simulink library "ASEToolBox"  (R2025b)
settings: Solver=ode45  StartTime=0.0  StopTime=10.0  RelTol=1e-3  EnableMultiTasking=on
values from neighbouring files (symbols this model uses):
  dt = get_param(gcbh, 'g_output_datatype')    [maskSysComCallbacks_Receive.m]    (also in maskSysComCallbacks_Send.m = get_param(gcbh, 'g_input_datatype'))
undefined symbols (not defined in the file or in its folder): dCx, dCy, dCz, DiscIntNeverNeededParam, Discrete, dmassX, dmassY, dmassZ, dMx, dMy, dMz, dp, dp0, dp1, dp2, dp3, dspblkCoreblockFVToolHelper, gcbh, lmd_high, lmd_low, magnitude, Newton, p0, p1, p2, p3, p4, phi0, phi000, phi1, phi2, phi3, phi4, r1, r2, r3, r4, Raphson, theta0, theta1, theta2, theta3, theta4, Time, u0, u1, u2, u3, v0, v0_max, v0_min, v1, v111, v2, v222, v3, v333, v4, W1, w1 ... (+4)
libraries: simulink x38, etargetslib x28, simulink_extras x5, slpidlib x2, ctrlSharedLib x2, aerolibatmos2 x1, aerolibconvert2 x1, aerolibtransform2 x1, sharedtransform x1, dspstat3 x1, dspsolvers x1
(part 4 of 6)

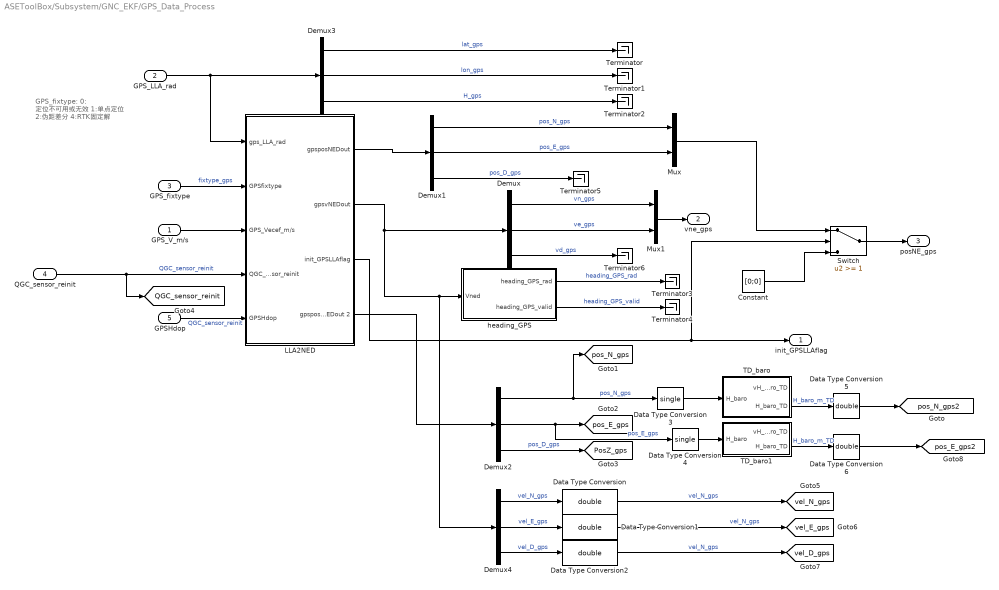
== system ASEToolBox/Subsystem/GNC_EKF/GPS_Data_Process ==
  note: GPS_fixtype:
      | 0: 定位不可用或无效
      | 1:单点定位
      | 2:伪距差分
      | 4:RTK固定解
  GPS_V_m/s : Inport
  GPS_LLA_rad : Inport  Port=2
  GPS_fixtype : Inport  Port=3
  QGC_sensor_reinit : Inport  Port=4
  GPSHdop : Inport  Port=5
  Constant : Constant  Value=[0;0]
  Data Type Conversion{,1..2,5..6} (5 alike) : DataTypeConversion  OutDataTypeStr=double  SaturateOnIntegerOverflow=off  RndMeth=Floor
  Data Type Conversion3 : DataTypeConversion  OutDataTypeStr=single  SaturateOnIntegerOverflow=off  RndMeth=Floor
  Data Type Conversion4 : DataTypeConversion  OutDataTypeStr=single  SaturateOnIntegerOverflow=off  RndMeth=Floor
  Demux{,1..4} (5 alike) : Demux  Outputs=3
  LLA2NED : Subsystem
  Mux : Mux  Inputs=2
  Mux1 : Mux  Inputs=2
  Switch : Switch  Threshold=1  SaturateOnIntegerOverflow=off  InputSameDT=off
  TD_baro : Subsystem
  TD_baro1 : Subsystem
  Terminator{,1..6} (7 alike) : Terminator
  heading_GPS : Subsystem
  init_GPSLLAflag : Outport
  vne_gps : Outport  Port=2
  posNE_gps : Outport  Port=3
  tag scope: PosZ_gps=global, QGC_sensor_reinit=global, pos_E_gps2=global, pos_E_gps=global, pos_N_gps2=global, pos_N_gps=global, vel_D_gps=global, vel_E_gps=global, vel_N_gps=global
  wires:
  GPS_fixtype/1 -> LLA2NED/2(GPSfixtype)  "fixtype_gps"
  Demux3/3 -> Terminator2/1  "H_gps"
  Demux/3 -> Terminator6/1  "vd_gps"
  Demux/1 -> Mux1/1  "vn_gps"
  GPS_LLA_rad/1 -> Demux3/1, LLA2NED/1(gps_LLA_rad)
  Demux/2 -> Mux1/2  "ve_gps"
  Demux3/2 -> Terminator1/1  "lon_gps"
  Demux3/1 -> Terminator/1  "lat_gps"
  QGC_sensor_reinit/1 -> [QGC_sensor_reinit], LLA2NED/4(QGC_sensor_reinit)  "QGC_sensor_reinit"
  LLA2NED/1("gpsposNEDout ") -> Demux1/1
  Demux1/1 -> Mux/1  "pos_N_gps"
  Demux1/2 -> Mux/2  "pos_E_gps"
  Demux1/3 -> Terminator5/1  "pos_D_gps"
  GPS_V_m/s/1 -> LLA2NED/3(GPS_Vecef_m/s)
  LLA2NED/2(gpsvNEDout) -> Demux4/1, heading_GPS/1(Vned), Demux/1
  heading_GPS/1(heading_GPS_rad) -> Terminator3/1  "heading_GPS_rad"
  heading_GPS/2(heading_GPS_valid) -> Terminator4/1  "heading_GPS_valid"
  Mux/1 -> Switch/1
  Mux1/1 -> vne_gps/1
  GPSHdop/1 -> LLA2NED/5(GPSHdop)  "QGC_sensor_reinit"
  LLA2NED/3(init_GPSLLAflag) -> Switch/2, init_GPSLLAflag/1
  Constant/1 -> Switch/3
  Switch/1 -> posNE_gps/1
  Demux2/1 -> [pos_N_gps], Data Type Conversion3/1  "pos_N_gps"
  Demux2/3 -> [PosZ_gps]  "pos_D_gps"
  Demux2/2 -> Data Type Conversion4/1, [pos_E_gps]  "pos_E_gps"
  LLA2NED/4(gpsposNEDout 2) -> Demux2/1
  Demux4/2 -> Data Type Conversion1/1  "vel_E_gps"
  Demux4/3 -> Data Type Conversion2/1  "vel_D_gps"
  Demux4/1 -> Data Type Conversion/1  "vel_N_gps"
  Data Type Conversion/1 -> [vel_N_gps]  "vel_N_gps"
  Data Type Conversion1/1 -> [vel_E_gps]  "vel_N_gps"
  Data Type Conversion2/1 -> [vel_D_gps]  "vel_N_gps"
  TD_baro/2(H_baro_TD) -> Data Type Conversion5/1  "H_baro_m_TD"
  TD_baro1/2(H_baro_TD) -> Data Type Conversion6/1  "H_baro_m_TD"
  Data Type Conversion3/1 -> TD_baro/1(H_baro)
  Data Type Conversion4/1 -> TD_baro1/1(H_baro)
  Data Type Conversion5/1 -> [pos_N_gps2]
  Data Type Conversion6/1 -> [pos_E_gps2]

== system ASEToolBox/Subsystem/GNC_EKF/Translation_estimate ==
  Cbn : Inport
  accl_ned_m/s2 : Inport  Port=2
  vne_gps : Inport  Port=3
  posNE_gps1 : Inport  Port=4
  GPSstate : Inport  Port=5
  GPSHdop : Inport  Port=6
  QGC_init : Inport  Port=7
  Enable : EnablePort
  Subsystem : Subsystem
  Subsystem2 : Subsystem
  V_Horizontal_estimation1 : Subsystem  Commented=on
  translate to N : Subsystem
  vxy_estimout : Outport
  Pxy_estimout : Outport  Port=2
  wires:
  Cbn/1 -> translate to N/1(Cbn)
  accl_ned_m/s2/1 -> translate to N/2(accl_ned)
  QGC_init/1 -> Subsystem/4(QGC_init), Subsystem2/3(QGC_init)
  posNE_gps1/1 -> Subsystem/2(pxy_GPS)
  GPSHdop/1 -> Subsystem2/4(DOP), Subsystem/5(DOP)
  Subsystem/1(pxy_est) -> Pxy_estimout/1
  Subsystem2/1(vxy_est) -> vxy_estimout/1, Subsystem/1(vxy)
  translate to N/1(accel_Horizontal_predict) -> Subsystem2/1(axy)
  vne_gps/1 -> Subsystem2/2(vxy_GPS)
  Subsystem2/2(GPSv_enable) -> Subsystem/3(GPSv_enable)

== system ASEToolBox/ACEModule/IMU/Subsystem5/Subsystem ==
  In1 : Inport
  Enable : EnablePort
  Byte Unpack1 : etargetslib/Byte Unpack  dimensions={6}  datatypes={'single'}  byteAlign=1
      settings: LibrarySourceBlock=embeddedtargetslib/Host Communication/Byte Unpack
  Out1 : Outport
  wires:
  In1/1 -> Byte Unpack1/1
  Byte Unpack1/1 -> Out1/1

== system ASEToolBox/ACEModule/ServoCardUnpack/Subsystem6/Subsystem ==
  In1 : Inport
  Enable : EnablePort
  Byte Unpack1 : etargetslib/Byte Unpack  dimensions={7}  datatypes={'single'}  byteAlign=1
      settings: LibrarySourceBlock=embeddedtargetslib/Host Communication/Byte Unpack
  Out1 : Outport
  wires:
  In1/1 -> Byte Unpack1/1
  Byte Unpack1/1 -> Out1/1

== system ASEToolBox/Aerocraft Model/ACE Equation of 6DOF's Motion/ACE Centroid Motion/231 Motion Subsystem ==
  F_All/m : Inport
  Deal with zero1 : Subsystem
  Deal with zero2 : Subsystem
  Deal with zero3 : Subsystem
  Demux1 : Demux  Outputs=3
  Discrete-Time Integrator : DiscreteIntegrator  InitialCondition=17.45  SampleTime=-1  ICPrevOutput=DiscIntNeverNeededParam  ICPrevScaledInput=DiscIntNeverNeededParam
  Discrete-Time Integrator1 : DiscreteIntegrator  SampleTime=-1  ICPrevOutput=DiscIntNeverNeededParam  ICPrevScaledInput=DiscIntNeverNeededParam
  Discrete-Time Integrator2 : DiscreteIntegrator  InitialCondition=60*pi/180  SampleTime=-1  ICPrevOutput=DiscIntNeverNeededParam  ICPrevScaledInput=DiscIntNeverNeededParam
  Gain6 : Gain  Gain=-1
  Integrator1 : Integrator  Commented=on  InitialCondition=17.45
  Integrator2 : Integrator  Commented=on  InitialCondition=60*pi/180
  Integrator3 : Integrator  Commented=on
  Product8 : Product  Inputs=/*  SaturateOnIntegerOverflow=on  OutDataTypeStr=Inherit: Same as first input
  Product9 : Product  Inputs=//*  SaturateOnIntegerOverflow=on  OutDataTypeStr=Inherit: Same as first input
  cosine1 : Trigonometry  Operator=cos
  V : Outport
  theta : Outport  Port=2
  sigma : Outport  Port=3
  wires:
  Discrete-Time Integrator1/1 -> sigma/1
  Discrete-Time Integrator2/1 -> cosine1/1, theta/1
  Discrete-Time Integrator/1 -> V/1, Deal with zero3/1(In1), Deal with zero1/1(In1)
  Gain6/1 -> Product9/3
  Deal with zero3/1(Out1) -> Product9/2
  Deal with zero2/1(Out1) -> Product9/1
  Product8/1 -> Discrete-Time Integrator2/1
  F_All/m/1 -> Demux1/1
  Demux1/1 -> Discrete-Time Integrator/1
  Demux1/3 -> Gain6/1
  Product9/1 -> Discrete-Time Integrator1/1
  Demux1/2 -> Product8/2
  cosine1/1 -> Deal with zero2/1(In1)
  Deal with zero1/1(Out1) -> Product8/1

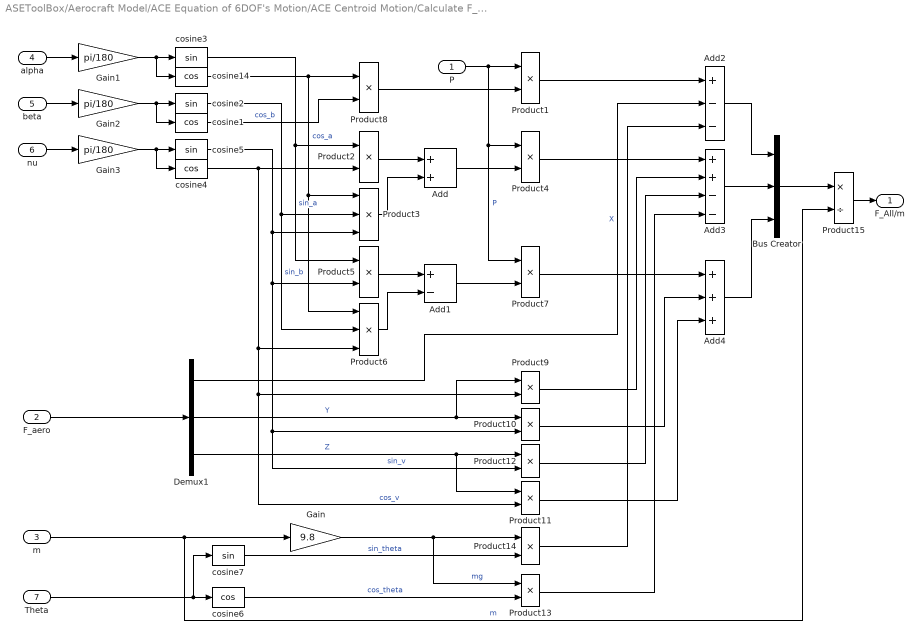
== system ASEToolBox/Aerocraft Model/ACE Equation of 6DOF's Motion/ACE Centroid Motion/Calculate F_all ==
  P : Inport
  F_aero : Inport  Port=2
  m : Inport  Port=3
  alpha : Inport  Port=4
  beta : Inport  Port=5
  nu : Inport  Port=6
  Theta : Inport  Port=7
  Add : Sum
  Add1 : Sum  Inputs=+-
  Add2 : Sum  Inputs=+--
  Add3 : Sum  Inputs=++--
  Add4 : Sum  Inputs=+++
  Bus Creator : BusCreator  Inputs=3
  Demux1 : Demux  Outputs=3
  Gain : Gain  Gain=9.8
  Gain1 : Gain  Gain=pi/180
  Gain2 : Gain  Gain=pi/180
  Gain3 : Gain  Gain=pi/180
  Product{1..2,4..5,7..14} (12 alike) : Product  Inputs=**  SaturateOnIntegerOverflow=on  OutDataTypeStr=Inherit: Same as first input
  Product15 : Product  Inputs=*/  SaturateOnIntegerOverflow=on  OutDataTypeStr=Inherit: Same as first input
  Product3 : Product  Inputs=***  SaturateOnIntegerOverflow=on  OutDataTypeStr=Inherit: Same as first input
  Product6 : Product  Inputs=***  SaturateOnIntegerOverflow=on  OutDataTypeStr=Inherit: Same as first input
  cosine{1,4,6,14} (4 alike) : Trigonometry  Operator=cos
  cosine{2..3,5,7} (4 alike) : Trigonometry
  F_All/m : Outport
  wires:
  F_aero/1 -> Demux1/1
  alpha/1 -> Gain1/1
  beta/1 -> Gain2/1
  nu/1 -> Gain3/1
  cosine14/1 -> Product8/1, Product3/1, Product6/1  "cos_a"
  cosine1/1 -> Product8/2  "cos_b"
  Product8/1 -> Product1/2
  P/1 -> Product1/1, Product4/1, Product7/1  "P"
  cosine4/1 -> Product2/2, Product6/3, Product9/2, Product11/2  "cos_v"
  cosine3/1 -> Product2/1, Product5/1  "sin_a"
  cosine2/1 -> Product3/2, Product6/2  "sin_b"
  cosine5/1 -> Product3/3, Product5/2, Product10/2, Product12/2  "sin_v"
  Product2/1 -> Add/1
  Product3/1 -> Add/2
  Add/1 -> Product4/2
  Product5/1 -> Add1/1
  Product6/1 -> Add1/2
  Add1/1 -> Product7/2
  Demux1/2 -> Product9/1, Product10/1  "Y"
  Demux1/3 -> Product12/1, Product11/1  "Z"
  m/1 -> Gain/1, Product15/2  "m"
  cosine7/1 -> Product14/2  "sin_theta"
  cosine6/1 -> Product13/2  "cos_theta"
  Product1/1 -> Add2/1
  Demux1/1 -> Add2/2  "X"
  Product14/1 -> Add2/3
  Product4/1 -> Add3/1
  Product9/1 -> Add3/2
  Product12/1 -> Add3/3
  Product13/1 -> Add3/4
  Product7/1 -> Add4/1
  Gain/1 -> Product14/1, Product13/1  "mg"
  Product10/1 -> Add4/2
  Product11/1 -> Add4/3
  Add2/1 -> Bus Creator/1
  Add3/1 -> Bus Creator/2
  Add4/1 -> Bus Creator/3
  Bus Creator/1 -> Product15/1
  Product15/1 -> F_All/m/1
  Theta/1 -> cosine6/1, cosine7/1
  Gain1/1 -> cosine3/1, cosine14/1
  Gain2/1 -> cosine2/1, cosine1/1
  Gain3/1 -> cosine5/1, cosine4/1

== system ASEToolBox/Aerocraft Model/ACE Equation of 6DOF's Motion/ACE Centroid Motion/Calculate xyz ==
  V : Inport
  theta : Inport  Port=2
  sigma : Inport  Port=3
  Discrete-Time Integrator : DiscreteIntegrator  SampleTime=-1  ICPrevOutput=DiscIntNeverNeededParam  ICPrevScaledInput=DiscIntNeverNeededParam
  Discrete-Time Integrator1 : DiscreteIntegrator  InitialCondition=0.001  SampleTime=-1  ICPrevOutput=DiscIntNeverNeededParam  ICPrevScaledInput=DiscIntNeverNeededParam
  Discrete-Time Integrator2 : DiscreteIntegrator  SampleTime=-1  ICPrevOutput=DiscIntNeverNeededParam  ICPrevScaledInput=DiscIntNeverNeededParam
  Mux1 : Mux  Inputs=3
  Mux2 : Mux  Inputs=3
  Vx : Product  Inputs=***  SaturateOnIntegerOverflow=on  OutDataTypeStr=Inherit: Same as first input
  Vy : Product  Inputs=**  SaturateOnIntegerOverflow=on  OutDataTypeStr=Inherit: Same as first input
  Vz : Gain  Gain=-1
  Vz. : Product  Inputs=***  SaturateOnIntegerOverflow=on  OutDataTypeStr=Inherit: Same as first input
  cosine10 : Trigonometry
  cosine11 : Trigonometry  Operator=cos
  cosine12 : Trigonometry  Operator=cos
  cosine14 : Trigonometry  Operator=cos
  cosine3 : Trigonometry
  x1 : Integrator  Commented=on
  y1 : Integrator  Commented=on  InitialCondition=0.001
  z1 : Integrator  Commented=on
  Vxyz : Outport
  xyz : Outport  Port=2
  wires:
  Discrete-Time Integrator2/1 -> Mux2/3
  Discrete-Time Integrator1/1 -> Mux2/2
  Discrete-Time Integrator/1 -> Mux2/1
  cosine10/1 -> Vz./3
  cosine14/1 -> Vz./2
  Vz/1 -> Mux1/3, Discrete-Time Integrator2/1  "vz"
  Vz./1 -> Vz/1
  Vy/1 -> Mux1/2, Discrete-Time Integrator1/1  "vy"
  Vx/1 -> Mux1/1, Discrete-Time Integrator/1  "vx"
  V/1 -> Vz./1, Vy/1, Vx/1
  Mux2/1 -> xyz/1
  Mux1/1 -> Vxyz/1
  cosine12/1 -> Vx/2
  cosine11/1 -> Vx/3
  cosine3/1 -> Vy/2
  theta/1 -> cosine14/1, cosine3/1, cosine11/1  "rad"
  sigma/1 -> cosine10/1, cosine12/1  "rad"

== system ASEToolBox/Aerocraft Model/ACE Equation of 6DOF's Motion/ACE Rotation Motion/Attitude Dynamic  ==
  note: d( w_x ) = M_x + (I_y-I_z)*w_y*w_z)
      |
      |  / I_x
      | .
  note: d( w_y ) = M_y + (I_z-I_x)*w_x*w_z)
      |
      |  / I_y
      | .
  note: d( w_z ) = M_z + (I_x-I_y)*w_x*w_y)
      |
      |  / I_z
      | .
  note: rad/s
  Mxyz : Inport
  Ixyz : Inport  Port=2
  Mux8 : Mux  Inputs=3
  Omega_Tx1 Subsystem : Subsystem
  Omega_Tx1 Subsystem1 : Subsystem
  Omega_Tx1 Subsystem2 : Subsystem
  Wxyz : Outport
  wires:
  Mxyz/1 -> Omega_Tx1 Subsystem/3(Mxyz), Omega_Tx1 Subsystem1/3(Mxyz), Omega_Tx1 Subsystem2/3(Mxyz)
  Mux8/1 -> Wxyz/1, Omega_Tx1 Subsystem/1(Wxyz), Omega_Tx1 Subsystem1/1(Wxyz), Omega_Tx1 Subsystem2/1(Wxyz)
  Omega_Tx1 Subsystem/1(Wx) -> Mux8/1
  Omega_Tx1 Subsystem1/1(Wy) -> Mux8/2
  Omega_Tx1 Subsystem2/1(Wz) -> Mux8/3
  Ixyz/1 -> Omega_Tx1 Subsystem/2(Ixyz), Omega_Tx1 Subsystem1/2(Ixyz), Omega_Tx1 Subsystem2/2(Ixyz)

== system ASEToolBox/Aerocraft Model/ACE Equation of 6DOF's Motion/ACE Rotation Motion/calculate Eular 231 ==
  note: d \phi = W_y * sin \gamma + W_z * cos \gamma
      |
      | d \psi = (W_y * cos \gamma - W_z * sin \gamma ) / cos \phi
      |
      | d \gamma = W_x  - tan \phi * ( W_y * cos \gamma - W_z * sin \gamma )
  Wxyz : Inport
  Eular0(deg) : Inport  Port=2
  Gain1 : Gain  Gain=pi/180
  Mux1 : Mux  Inputs=3
  PhiPsiGam : Gain  Gain=180/pi
  gam Subsystem : Subsystem
  phi Subsystem : Subsystem
  psi Subsystem : Subsystem
  Eular(deg) : Outport
  wires:
  Gain1/1 -> phi Subsystem/3(Eular0), psi Subsystem/3(Eular0), gam Subsystem/3(Eular0)
  PhiPsiGam/1 -> Eular(deg)/1
  Eular0(deg)/1 -> Gain1/1
  Mux1/1 -> PhiPsiGam/1, gam Subsystem/1(Eular), psi Subsystem/1(Eular), phi Subsystem/1(Eular)
  gam Subsystem/1(gam) -> Mux1/3
  psi Subsystem/1(psi) -> Mux1/2
  Wxyz/1 -> gam Subsystem/2(Wxyz), psi Subsystem/2(Wxyz), phi Subsystem/2(Wxyz)
  phi Subsystem/1(phi) -> Mux1/1

== system ASEToolBox/Aerocraft Model/ACE Equation of 6DOF's Motion/Aero Force & Moment/ACE Aerodynamic for 6DOF ==
  Ma : Inport
  abv : Inport  Port=2
  WXYZ : Inport  Port=3
  DeltXYZ : Inport  Port=4
  CD : Lookup2D  RowIndex=[-2 -1 0.5 1 2 3 4 5 6 7 8 9 10]  ColumnIndex=[0.3 0.4 0.5 0.6 0.7 0.8]  Table=|  SaturateOnIntegerOverflow=off  InputSameDT=off
      | [0.184400000000000	0.176300000000000	0.168500000000000	0.162600000000000	0.158700000000000	0.154800000000000
      | 0.194000000000000	0.185600000000000	0.177400000000000	0.171100000000000	0.166800000000000	0.162200000000000
      | 0.196300000000000	0.187800000000000	0.179600000000000	0.173200000000000	0.168700000000000	0.164000000000000
      | 0.194000000000000	0.185600000000000	0.177400000000000	0.171100000000000	0.166800000000000	0.162200000000000
      | 0.184400000000000	0.176300000000000	0.168500000000000	0.162600000000000	0.158700000000000	0.154800000000000
      | 0.168000000000000	0.160300000000000	0.153000000000000	0.147900000000000	0.144800000000000	0.141900000000000
      | 0.144500000000000	0.137300000000000	0.130800000000000	0.126700000000000	0.124700000000000	0.123200000000000
      | 0.113500000000000	0.107100000000000	0.101600000000000	0.0987000000000000	0.0982000000000000	0.0985000000000000
      | 0.0748000000000000	0.0694000000000000	0.0651000000000000	0.0637000000000000	0.0650000000000000	0.0674000000000000
      | 0.0284000000000000	0.0241000000000000	0.0212000000000000	0.0217000000000000	0.0250000000000000	0.0300000000000000
      | -0.0258000000000000	-0.0289000000000000	-0.0302000000000000	-0.0276000000000000	-0.0220000000000000	-0.0140000000000000
      | -0.0878000000000000	-0.0895000000000000	-0.0890000000000000	-0.0841000000000000	-0.0758000000000000	-0.0646000000000000
      | -0.157700000000000	-0.157800000000000	-0.155300000000000	-0.147900000000000	-0.136600000000000	-0.121800000000000
      | ]
  CL Subsystem : Subsystem
  CZ Subsystem : Subsystem
  Mux : Mux  Inputs=3
  Mux1 : Mux  Inputs=3
  Mx Subsystem : Subsystem
  My Subsystem : Subsystem
  Mz Subsystem : Subsystem
  Selector : Selector  InputPortWidth=3  IndexOptions=Index vector (dialog)  Indices=[1]  OutputSizes=1
  Selector1 : Selector  InputPortWidth=3  IndexOptions=Index vector (dialog)  Indices=[2]  OutputSizes=1
  Selector2 : Selector  InputPortWidth=3  IndexOptions=Index vector (dialog)  Indices=[1]  OutputSizes=1
  Selector3 : Selector  InputPortWidth=3  IndexOptions=Index vector (dialog)  Indices=[1]  OutputSizes=1
  Selector4 : Selector  InputPortWidth=3  IndexOptions=Index vector (dialog)  Indices=[2]  OutputSizes=1
  Selector5 : Selector  InputPortWidth=3  IndexOptions=Index vector (dialog)  Indices=3  OutputSizes=1
  Selector6 : Selector  InputPortWidth=3  IndexOptions=Index vector (dialog)  Indices=3  OutputSizes=1
  Cxyz : Outport
  Mxyz : Outport  Port=2
  wires:
  Selector6/1 -> Mz Subsystem/3(DeltZ), CL Subsystem/3(DeltZ)  "DeltZ"
  Selector5/1 -> Mz Subsystem/4(WZ)  "WZ"
  Selector4/1 -> Mx Subsystem/6(WY), My Subsystem/3(WY)  "WY"
  Selector3/1 -> My Subsystem/2(WX), Mx Subsystem/5(WX)  "WX"
  Selector2/1 -> Mx Subsystem/4(DeltX)  "DeltX"
  WXYZ/1 -> Selector5/1, Selector4/1, Selector3/1
  DeltXYZ/1 -> Selector6/1, Selector2/1
  Mz Subsystem/1(Mz) -> Mux1/3
  Ma/1 -> Mz Subsystem/1(Ma), My Subsystem/4(Ma), Mx Subsystem/2(Ma), CZ Subsystem/3(Ma), CL Subsystem/2(Ma), CD/2  "Ma"
  abv/1 -> Selector/1, Selector1/1
  CD/1 -> Mux/1
  CL Subsystem/1(CL) -> Mux/2
  CZ Subsystem/1(CZ) -> Mux/3
  Mux/1 -> Cxyz/1
  Mx Subsystem/1(Mx) -> Mux1/1
  My Subsystem/1(My) -> Mux1/2
  Mux1/1 -> Mxyz/1
  Selector/1 -> Mz Subsystem/2(alpha), My Subsystem/5(alpha), Mx Subsystem/3(alpha), CZ Subsystem/2(alpha), CL Subsystem/1(alpha), CD/1  "alpha"
  Selector1/1 -> My Subsystem/1(Beta), Mx Subsystem/1(Beta), CZ Subsystem/1(beta)  "beta"

== system ASEToolBox/Aerocraft Model/ACE Equation of 6DOF's Motion/Aero Force & Moment/Subsystem ==
  XYZ : Inport
  dmassXYZ : Inport  Port=2
  L : Inport  Port=3
  Add1 : Sum  Inputs=+-
  Add2 : Sum  Inputs=+-
  Add4 : Sum
  Demux1 : Demux  Outputs=3
  Demux2 : Demux  Outputs=3
  Mux3 : Mux  Inputs=3
  Product{3..7,9..10} (7 alike) : Product  Inputs=**  SaturateOnIntegerOverflow=on  OutDataTypeStr=Inherit: Same as first input
  Selector1 : Selector  InputPortWidth=3  IndexOptions=Index vector (dialog)  Indices=[3 2 1]  OutputSizes=1
  dMxyz : Outport
  wires:
  Selector1/1 -> dMxyz/1
  dmassXYZ/1 -> Demux1/1
  Product3/1 -> Selector1/1
  L/1 -> Product3/2
  XYZ/1 -> Demux2/1
  Mux3/1 -> Product3/1
  Demux2/3 -> Product9/1, Product7/1  "Z"
  Demux1/3 -> Product10/2, Product6/2  "dz"
  Demux1/1 -> Product7/2, Product5/2  "dx"
  Demux2/2 -> Product10/1, Product5/1  "Y"
  Demux1/2 -> Product9/2, Product4/2  "dy"
  Demux2/1 -> Product6/1, Product4/1  "X"
  Add2/1 -> Mux3/3
  Product10/1 -> Add2/2
  Product9/1 -> Add2/1
  Add1/1 -> Mux3/2
  Product7/1 -> Add1/2
  Product6/1 -> Add1/1
  Add4/1 -> Mux3/1
  Product5/1 -> Add4/2
  Product4/1 -> Add4/1

== system ASEToolBox/Aerocraft Model/ACE Equation of 6DOF's Motion/Aero Force & Moment/q Subsystem ==
  V : Inport
  Density : Inport  Port=2
  Gain : Gain  Gain=0.5
  Product : Product  RndMeth=Zero
  U2 : Math  Operator=square  SignedPower=on
  q : Outport
  wires:
  Product/1 -> q/1
  V/1 -> U2/1
  Density/1 -> Product/1
  U2/1 -> Gain/1
  Gain/1 -> Product/2

== system ASEToolBox/Aerocraft Model/ACE Equation of 6DOF's Motion/Constraint Equation2/alpha Subsystem ==
  note: 231
      |
      | sin\beta = cos\theta * [ cos\gamma * sin(\psi - \sigma) + sin\phi * sin\gamma * cos(\psi - \sigma) ] - sin\theta * cos\phi * sin\gamma
      |
      | sin\alpha * cos\beta = cos\theta * [ sin\phi * cos\gamma * cos(\psi - \sigma) - sin\gamma * sin(\psi - \sigma) ] - sin\theta * cos\phi * cos\gamma
      |
      | sin\nu * cos\theta = cos\alpha * sin\beta * sin\phi - sin\alpha * sin\beta * cos\gamma * cos\phi + cos\beta * sin\gamma * cos\phi
      | .
  theta : Inport
  sigma : Inport  Port=2
  Eular : Inport  Port=3
  beta : Inport  Port=4
  Demux3 : Demux  Outputs=3
  Divide : Product  Inputs=***
  Divide1 : Product  Inputs=*/
  Divide2 : Product  Inputs=**
  Divide3 : Product  Inputs=**
  Divide4 : Product  Inputs=***
  Subtract : Sum  Inputs=-+
  Subtract1 : Sum  Inputs=+-
  Subtract2 : Sum  Inputs=+-
  Trigonometric Function{1,4..5,10,15} (5 alike) : Trigonometry  Operator=cos
  Trigonometric Function{3,13..14,16} (4 alike) : Trigonometry
  Trigonometric Function2 : Trigonometry  Operator=asin
  alpha : Outport
  wires:
  Trigonometric Function5/1 -> Divide3/2
  Subtract1/1 -> Divide3/1
  Subtract2/1 -> Divide1/1
  Trigonometric Function4/1 -> Divide/3, Divide4/2
  Divide4/1 -> Subtract2/2
  Divide3/1 -> Subtract2/1
  Trigonometric Function14/1 -> Divide4/3
  Trigonometric Function15/1 -> Divide4/1
  Trigonometric Function13/1 -> Divide2/1
  Trigonometric Function3/1 -> Divide2/2
  Divide2/1 -> Subtract1/2
  Trigonometric Function16/1 -> Divide/2
  Trigonometric Function10/1 -> Divide/1
  Demux3/1 -> Trigonometric Function15/1, Trigonometric Function16/1  "phi"
  Subtract/1 -> Trigonometric Function13/1, Trigonometric Function10/1
  Demux3/2 -> Subtract/2  "psi"
  sigma/1 -> Subtract/1
  theta/1 -> Trigonometric Function5/1, Trigonometric Function14/1
  Eular/1 -> Demux3/1
  Demux3/3 -> Trigonometric Function3/1, Trigonometric Function4/1  "gamma"
  Divide/1 -> Subtract1/1
  beta/1 -> Trigonometric Function1/1
  Trigonometric Function1/1 -> Divide1/2
  Divide1/1 -> Trigonometric Function2/1
  Trigonometric Function2/1 -> alpha/1

== system ASEToolBox/Aerocraft Model/ACE Equation of 6DOF's Motion/Constraint Equation2/beta Subsystem ==
  note: 231
      |
      | sin\beta = cos\theta * [ cos\gamma * sin(\psi - \sigma) + sin\phi * sin\gamma * cos(\psi - \sigma) ] - sin\theta * cos\phi * sin\gamma
      |
      | sin\alpha * cos\beta = cos\theta * [ sin\phi * cos\gamma * cos(\psi - \sigma) - sin\gamma * sin(\psi - \sigma) ] - sin\theta * cos\phi * cos\gamma
      |
      | sin\nu * cos\theta = cos\alpha * sin\beta * sin\phi - sin\alpha * sin\beta * cos\gamma * cos\phi + cos\beta * sin\gamma * cos\phi
      | .
  theta : Inport
  sigma : Inport  Port=2
  Eular : Inport  Port=3
  Demux3 : Demux  Outputs=3
  Divide : Product  Inputs=***
  Divide1 : Product  Inputs=**
  Divide2 : Product  Inputs=**
  Divide3 : Product  Inputs=***
  Subtract : Sum  Inputs=-+
  Subtract1 : Sum  Inputs=+-
  Subtract2 : Sum
  Trigonometric Function1 : Trigonometry  Operator=asin
  Trigonometric Function{10..11,13,15} (4 alike) : Trigonometry  Operator=cos
  Trigonometric Function{9,12,14,16} (4 alike) : Trigonometry
  beta : Outport
  wires:
  Eular/1 -> Demux3/1
  theta/1 -> Trigonometric Function14/1, Trigonometric Function13/1
  sigma/1 -> Subtract/1
  Demux3/2 -> Subtract/2  "psi"
  Subtract/1 -> Trigonometric Function9/1, Trigonometric Function10/1
  Demux3/3 -> Trigonometric Function12/1, Trigonometric Function11/1  "gamma"
  Trigonometric Function10/1 -> Divide/1
  Demux3/1 -> Trigonometric Function16/1, Trigonometric Function15/1  "phi"
  Trigonometric Function12/1 -> Divide/3, Divide3/3  "sin\\gamma"
  Trigonometric Function9/1 -> Divide1/1
  Trigonometric Function11/1 -> Divide1/2
  Trigonometric Function16/1 -> Divide/2
  Divide1/1 -> Subtract2/1
  Divide/1 -> Subtract2/2
  Subtract2/1 -> Divide2/2
  Trigonometric Function13/1 -> Divide2/1
  Trigonometric Function14/1 -> Divide3/1  "sin\\theta"
  Trigonometric Function15/1 -> Divide3/2
  Divide2/1 -> Subtract1/1
  Divide3/1 -> Subtract1/2
  Subtract1/1 -> Trigonometric Function1/1
  Trigonometric Function1/1 -> beta/1  "rad"

== system ASEToolBox/Aerocraft Model/ACE Equation of 6DOF's Motion/Constraint Equation2/nu Subsystem ==
  note: 231
      |
      | sin\beta = cos\theta * [ cos\gamma * sin(\psi - \sigma) + sin\phi * sin\gamma * cos(\psi - \sigma) ] - sin\theta * cos\phi * sin\gamma
      |
      | sin\alpha * cos\beta = cos\theta * [ sin\phi * cos\gamma * cos(\psi - \sigma) - sin\gamma * sin(\psi - \sigma) ] - sin\theta * cos\phi * cos\gamma
      |
      | sin\nu * cos\theta = cos\alpha * sin\beta * sin\phi - sin\alpha * sin\beta * cos\gamma * cos\phi + cos\beta * sin\gamma * cos\phi
      | .
  alpha : Inport
  beta : Inport  Port=2
  theta : Inport  Port=3
  Eular : Inport  Port=4
  Demux3 : Demux  Outputs=3
  Divide1 : Product  Inputs=*/
  Divide2 : Product  Inputs=****
  Divide3 : Product  Inputs=***
  Divide4 : Product  Inputs=***
  Subtract2 : Sum  Inputs=+-+
  Terminator : Terminator
  Trigonometric Function{1..2,4,6,9} (5 alike) : Trigonometry  Operator=cos
  Trigonometric Function{3,7..8,15} (4 alike) : Trigonometry
  Trigonometric Function5 : Trigonometry  Operator=asin
  nu : Outport
  wires:
  Divide3/1 -> Subtract2/3
  Trigonometric Function8/1 -> Divide3/2  "sin\\gamma"
  Trigonometric Function9/1 -> Divide3/3  "cos\\beta"
  Divide2/1 -> Subtract2/2
  Trigonometric Function4/1 -> Divide3/1, Divide2/3  "cos\\phi"
  Trigonometric Function2/1 -> Divide2/4  "cos\\gamma"
  Trigonometric Function3/1 -> Divide2/1  "sin\\alpha"
  Divide4/1 -> Subtract2/1
  Demux3/2 -> Terminator/1  "psi"
  Trigonometric Function15/1 -> Divide4/3  "sin\\phi"
  Trigonometric Function7/1 -> Divide2/2, Divide4/2  "sin\\beta"
  Trigonometric Function6/1 -> Divide4/1  "cos\\alpha"
  beta/1 -> Trigonometric Function9/1, Trigonometric Function7/1
  alpha/1 -> Trigonometric Function3/1, Trigonometric Function6/1
  theta/1 -> Trigonometric Function1/1
  Trigonometric Function5/1 -> nu/1  "rad"
  Trigonometric Function1/1 -> Divide1/2
  Eular/1 -> Demux3/1
  Demux3/1 -> Trigonometric Function4/1, Trigonometric Function15/1  "phi"
  Demux3/3 -> Trigonometric Function8/1, Trigonometric Function2/1  "gamma"
  Subtract2/1 -> Divide1/1
  Divide1/1 -> Trigonometric Function5/1

== system ASEToolBox/SIMSystemModule/ASEMonitorIn/Subsystem1/Subsystem ==
  In1 : Inport
  Enable : EnablePort
  Byte Unpack1 : etargetslib/Byte Unpack  dimensions={g_iVarNum}  datatypes={'single'}  byteAlign=1
      settings: LibrarySourceBlock=embeddedtargetslib/Host Communication/Byte Unpack
  Out1 : Outport
  wires:
  Byte Unpack1/1 -> Out1/1
  In1/1 -> Byte Unpack1/1

== system ASEToolBox/Subsystem/Formation-Control/Consistent formation control /一致性控制——F1 ==
  u0_k : Inport
  X0_k_1 : Inport  Port=2
  X1_k_1 : Inport  Port=3
  X2_k_1 : Inport  Port=4
  dp : Inport  Port=5
  Add{,1..2,4..5,8} (6 alike) : Sum  Inputs=+-
  Add3 : Sum  Inputs=-+
  Add6 : Sum  Inputs=+++
  Add7 : Sum  Inputs=+--
  Bus Selector : BusSelector  OutputSignals=p1_k_1
  Bus Selector1 : BusSelector  OutputSignals=p2_k_1
  Bus Selector2 : BusSelector  OutputSignals=p0_k_1
  Bus Selector3 : BusSelector  OutputSignals=dp1,dp0
  Bus Selector4 : BusSelector  OutputSignals=dp1,dp2
  Bus Selector5 : BusSelector  OutputSignals=v111_k_1
  Bus Selector6 : BusSelector  OutputSignals=v000_k_1
  Demux1 : Demux  Outputs=3
  Gain : Gain  Gain=2
  Gain1 : Gain  Gain=0.5
  Gain2 : Gain  Gain=2
  MATLAB Function1 : MATLAB Function  TreatAsAtomicUnit=on
  MATLAB Function2 : MATLAB Function  TreatAsAtomicUnit=on
  MATLAB Function4 : MATLAB Function  TreatAsAtomicUnit=on
  Mux : Mux  Inputs=3
  Subsystem1 : Subsystem
  X0_k_1_2 : InportShadow  Port=2
  X1_k_1_1 : InportShadow  Port=3
  dp1 : InportShadow  Port=5
  u1_k : Outport
  wires:
  Gain2/1 -> Add8/2
  Add3/1 -> Add6/2
  Bus Selector5/1 -> Add7/1  "<v111_k_1>"
  Bus Selector/1 -> Add/1, Add1/1  "<p1_k_1>"
  X0_k_1_2/1 -> Bus Selector2/1
  X2_k_1/1 -> Bus Selector1/1
  Bus Selector4/1 -> Add4/1  "<dp1>"
  X1_k_1_1/1 -> Bus Selector5/1
  Gain1/1 -> Demux1/1  "控制量z"
  Add6/1 -> Gain1/1
  Bus Selector6/1 -> Add7/2  "<v000_k_1>"
  X1_k_1/1 -> Bus Selector/1
  Bus Selector3/1 -> Add2/1  "<dp1>"
  u0_k/1 -> Add8/1
  Bus Selector4/2 -> Add4/2  "<dp2>"
  Bus Selector3/2 -> Add2/2  "<dp0>"
  Add7/1 -> Gain2/1
  Add1/1 -> Add5/1
  Subsystem1/1(wxyz) -> Gain/1
  dp/1 -> Bus Selector3/1
  X0_k_1/1 -> Bus Selector6/1
  Mux/1 -> Add7/3
  Add4/1 -> Add5/2
  Add2/1 -> Add3/1
  Add5/1 -> Add6/3
  Bus Selector1/1 -> Add1/2  "<p2_k_1>"
  Add/1 -> Add3/2
  Gain/1 -> Add6/1
  Add8/1 -> u1_k/1
  dp1/1 -> Bus Selector4/1
  Bus Selector2/1 -> Add/2  "<p0_k_1>"
  MATLAB Function4/1(result) -> Mux/1
  MATLAB Function1/1(result) -> Mux/2
  Demux1/1 -> MATLAB Function4/1(r)
  Demux1/3 -> MATLAB Function2/1(r)
  Demux1/2 -> MATLAB Function1/1(r)
  MATLAB Function2/1(result) -> Mux/3

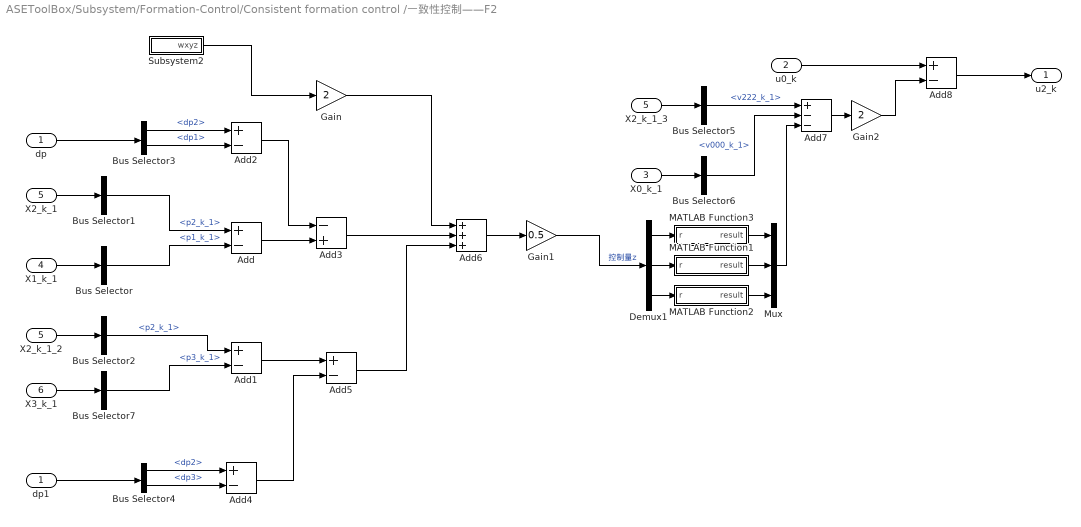
== system ASEToolBox/Subsystem/Formation-Control/Consistent formation control /一致性控制——F2 ==
  dp : Inport
  u0_k : Inport  Port=2
  X0_k_1 : Inport  Port=3
  X1_k_1 : Inport  Port=4
  X2_k_1 : Inport  Port=5
  X3_k_1 : Inport  Port=6
  Add{,1..2,4..5,8} (6 alike) : Sum  Inputs=+-
  Add3 : Sum  Inputs=-+
  Add6 : Sum  Inputs=+++
  Add7 : Sum  Inputs=+--
  Bus Selector : BusSelector  OutputSignals=p1_k_1
  Bus Selector1 : BusSelector  OutputSignals=p2_k_1
  Bus Selector2 : BusSelector  OutputSignals=p2_k_1
  Bus Selector3 : BusSelector  OutputSignals=dp2,dp1
  Bus Selector4 : BusSelector  OutputSignals=dp2,dp3
  Bus Selector5 : BusSelector  OutputSignals=v222_k_1
  Bus Selector6 : BusSelector  OutputSignals=v000_k_1
  Bus Selector7 : BusSelector  OutputSignals=p3_k_1
  Demux1 : Demux  Outputs=3
  Gain : Gain  Gain=2
  Gain1 : Gain  Gain=0.5
  Gain2 : Gain  Gain=2
  MATLAB Function1 : MATLAB Function  TreatAsAtomicUnit=on
  MATLAB Function2 : MATLAB Function  TreatAsAtomicUnit=on
  MATLAB Function3 : MATLAB Function  TreatAsAtomicUnit=on
  Mux : Mux  Inputs=3
  Subsystem2 : Subsystem
  X2_k_1_2 : InportShadow  Port=5
  X2_k_1_3 : InportShadow  Port=5
  dp1 : InportShadow
  u2_k : Outport
  wires:
  dp1/1 -> Bus Selector4/1
  Add8/1 -> u2_k/1
  Gain/1 -> Add6/1
  Add/1 -> Add3/2
  Add5/1 -> Add6/3
  Add2/1 -> Add3/1
  Add4/1 -> Add5/2
  Mux/1 -> Add7/3
  X0_k_1/1 -> Bus Selector6/1
  dp/1 -> Bus Selector3/1
  Subsystem2/1(wxyz) -> Gain/1
  Add1/1 -> Add5/1
  Add7/1 -> Gain2/1
  Bus Selector3/2 -> Add2/2  "<dp1>"
  u0_k/1 -> Add8/1
  X1_k_1/1 -> Bus Selector/1
  Bus Selector6/1 -> Add7/2  "<v000_k_1>"
  Add6/1 -> Gain1/1
  Gain1/1 -> Demux1/1  "控制量z"
  X2_k_1_3/1 -> Bus Selector5/1
  Bus Selector4/1 -> Add4/1  "<dp2>"
  X2_k_1/1 -> Bus Selector1/1
  Bus Selector5/1 -> Add7/1  "<v222_k_1>"
  Add3/1 -> Add6/2
  Gain2/1 -> Add8/2
  Bus Selector1/1 -> Add/1  "<p2_k_1>"
  Bus Selector/1 -> Add/2  "<p1_k_1>"
  Bus Selector2/1 -> Add1/1  "<p2_k_1>"
  X2_k_1_2/1 -> Bus Selector2/1
  X3_k_1/1 -> Bus Selector7/1
  Bus Selector7/1 -> Add1/2  "<p3_k_1>"
  Bus Selector3/1 -> Add2/1  "<dp2>"
  Bus Selector4/2 -> Add4/2  "<dp3>"
  Demux1/1 -> MATLAB Function3/1(r)
  Demux1/2 -> MATLAB Function1/1(r)
  Demux1/3 -> MATLAB Function2/1(r)
  MATLAB Function3/1(result) -> Mux/1
  MATLAB Function1/1(result) -> Mux/2
  MATLAB Function2/1(result) -> Mux/3

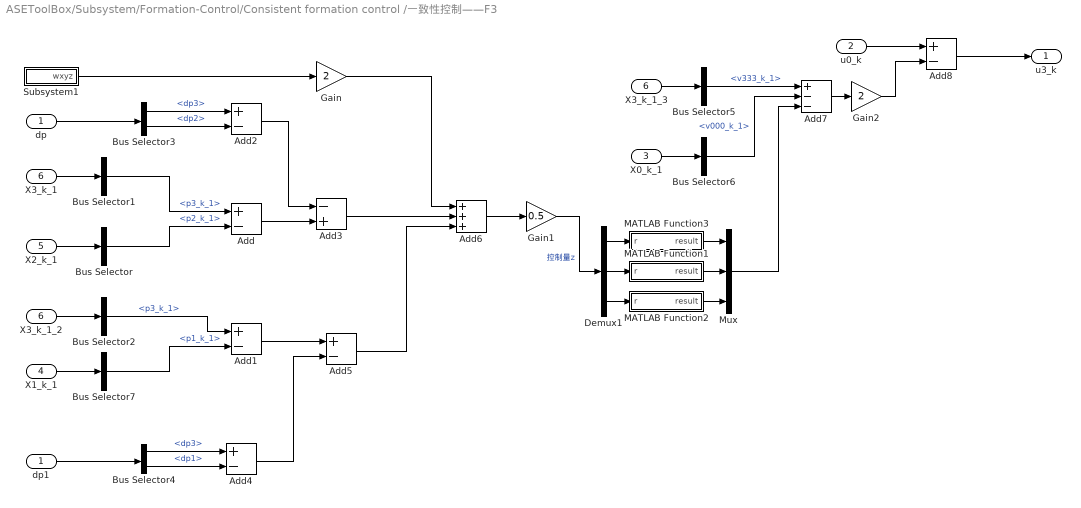
== system ASEToolBox/Subsystem/Formation-Control/Consistent formation control /一致性控制——F3 ==
  dp : Inport
  u0_k : Inport  Port=2
  X0_k_1 : Inport  Port=3
  X1_k_1 : Inport  Port=4
  X2_k_1 : Inport  Port=5
  X3_k_1 : Inport  Port=6
  Add{,1..2,4..5,8} (6 alike) : Sum  Inputs=+-
  Add3 : Sum  Inputs=-+
  Add6 : Sum  Inputs=+++
  Add7 : Sum  Inputs=+--
  Bus Selector : BusSelector  OutputSignals=p2_k_1
  Bus Selector1 : BusSelector  OutputSignals=p3_k_1
  Bus Selector2 : BusSelector  OutputSignals=p3_k_1
  Bus Selector3 : BusSelector  OutputSignals=dp3,dp2
  Bus Selector4 : BusSelector  OutputSignals=dp3,dp1
  Bus Selector5 : BusSelector  OutputSignals=v333_k_1
  Bus Selector6 : BusSelector  OutputSignals=v000_k_1
  Bus Selector7 : BusSelector  OutputSignals=p1_k_1
  Demux1 : Demux  Outputs=3
  Gain : Gain  Gain=2
  Gain1 : Gain  Gain=0.5
  Gain2 : Gain  Gain=2
  MATLAB Function1 : MATLAB Function  TreatAsAtomicUnit=on
  MATLAB Function2 : MATLAB Function  TreatAsAtomicUnit=on
  MATLAB Function3 : MATLAB Function  TreatAsAtomicUnit=on
  Mux : Mux  Inputs=3
  Subsystem1 : Subsystem
  X3_k_1_2 : InportShadow  Port=6
  X3_k_1_3 : InportShadow  Port=6
  dp1 : InportShadow
  u3_k : Outport
  wires:
  Bus Selector7/1 -> Add1/2  "<p1_k_1>"
  X3_k_1_2/1 -> Bus Selector2/1
  Bus Selector2/1 -> Add1/1  "<p3_k_1>"
  Bus Selector/1 -> Add/2  "<p2_k_1>"
  Bus Selector1/1 -> Add/1  "<p3_k_1>"
  Gain2/1 -> Add8/2
  Add3/1 -> Add6/2
  Bus Selector5/1 -> Add7/1  "<v333_k_1>"
  X3_k_1_3/1 -> Bus Selector5/1
  Gain1/1 -> Demux1/1  "控制量z"
  Add6/1 -> Gain1/1
  Bus Selector6/1 -> Add7/2  "<v000_k_1>"
  u0_k/1 -> Add8/1
  Add7/1 -> Gain2/1
  Add1/1 -> Add5/1
  dp/1 -> Bus Selector3/1
  X0_k_1/1 -> Bus Selector6/1
  Mux/1 -> Add7/3
  Add4/1 -> Add5/2
  Add2/1 -> Add3/1
  Add5/1 -> Add6/3
  Add/1 -> Add3/2
  Gain/1 -> Add6/1
  Add8/1 -> u3_k/1
  dp1/1 -> Bus Selector4/1
  X3_k_1/1 -> Bus Selector1/1
  X2_k_1/1 -> Bus Selector/1
  X1_k_1/1 -> Bus Selector7/1
  Bus Selector3/1 -> Add2/1  "<dp3>"
  Bus Selector3/2 -> Add2/2  "<dp2>"
  Bus Selector4/1 -> Add4/1  "<dp3>"
  Bus Selector4/2 -> Add4/2  "<dp1>"
  Subsystem1/1(wxyz) -> Gain/1
  MATLAB Function3/1(result) -> Mux/1
  MATLAB Function1/1(result) -> Mux/2
  Demux1/1 -> MATLAB Function3/1(r)
  Demux1/3 -> MATLAB Function2/1(r)
  Demux1/2 -> MATLAB Function1/1(r)
  MATLAB Function2/1(result) -> Mux/3

== system ASEToolBox/Subsystem/Formation-Control/Follower1/Subsystem ==
  v111_k_1 : Inport
  v000_k_1 : Inport  Port=2
  Abs : Abs  SaturateOnIntegerOverflow=off
  Abs1 : Abs  SaturateOnIntegerOverflow=off
  Abs2 : Abs  SaturateOnIntegerOverflow=off
  Add : Sum  Inputs=+-
  Add1 : Sum  Inputs=+-
  Add2 : Sum  Inputs=+-
  Demux : Demux  Outputs=3
  Demux1 : Demux  Outputs=3
  Max : MinMax  Function=max  Inputs=3
  Relational Operator : RelationalOperator  Operator=>  OutDataTypeStr=boolean  RndMeth=Simplest  InputSameDT=off
  get lmd : Subsystem
  order : Outport
  wires:
  v111_k_1/1 -> Demux/1
  v000_k_1/1 -> Demux1/1
  Demux/1 -> Add/1
  Demux1/1 -> Add/2
  Demux/2 -> Add1/1
  Demux1/2 -> Add1/2
  Demux1/3 -> Add2/2
  Demux/3 -> Add2/1
  Add/1 -> Abs/1
  Add1/1 -> Abs1/1
  Add2/1 -> Abs2/1
  Abs/1 -> Max/1
  Abs1/1 -> Max/2
  Abs2/1 -> Max/3
  Max/1 -> Relational Operator/1
  get lmd/1(lmd) -> Relational Operator/2
  Relational Operator/1 -> order/1

== system ASEToolBox/Subsystem/Formation-Control/Follower1/Subsystem1 ==
  Clock : Clock
  Constant : Constant
  Constant1 : Constant  Value=0
  Switch1 : Switch  Criteria=u2 > Threshold  Threshold=40  SaturateOnIntegerOverflow=off  InputSameDT=off
  Out1 : Outport
  wires:
  Clock/1 -> Switch1/2
  Constant/1 -> Switch1/1
  Constant1/1 -> Switch1/3
  Switch1/1 -> Out1/1

== system ASEToolBox/Subsystem/Formation-Control/Follower1/质心运动方程 ==
  v1 : Inport
  theta1 : Inport  Port=2
  phi1 : Inport  Port=3
  Enable : EnablePort
  Cos : Trigonometry  Operator=cos
  Cos1 : Trigonometry  Operator=cos
  Mux : Mux  Inputs=3
  Product : Product  Inputs=3
  Product1 : Product  Inputs=3
  Product2 : Product
  Sin : Trigonometry
  Sin1 : Trigonometry
  v111 : Outport
  wires:
  Sin1/1 -> Product2/1
  Mux/1 -> v111/1
  Product2/1 -> Mux/3
  Cos1/1 -> Product1/2, Product/2
  Sin/1 -> Product1/1
  Product1/1 -> Mux/2
  Product/1 -> Mux/1
  v1/1 -> Product/3, Product1/3, Product2/2
  Cos/1 -> Product/1
  phi1/1 -> Sin1/1, Cos1/1
  theta1/1 -> Sin/1, Cos/1

== system ASEToolBox/Subsystem/Formation-Control/Follower2/Subsystem ==
  v222_k_1 : Inport
  v000_k_1 : Inport  Port=2
  Abs : Abs  SaturateOnIntegerOverflow=off
  Abs1 : Abs  SaturateOnIntegerOverflow=off
  Abs2 : Abs  SaturateOnIntegerOverflow=off
  Add : Sum  Inputs=+-
  Add1 : Sum  Inputs=+-
  Add2 : Sum  Inputs=+-
  Demux : Demux  Outputs=3
  Demux1 : Demux  Outputs=3
  Max : MinMax  Function=max  Inputs=3
  Relational Operator : RelationalOperator  Operator=>  OutDataTypeStr=boolean  RndMeth=Simplest  InputSameDT=off
  get lmd : Subsystem
  order : Outport
  wires:
  Relational Operator/1 -> order/1
  get lmd/1(lmd) -> Relational Operator/2
  Max/1 -> Relational Operator/1
  Abs2/1 -> Max/3
  Abs1/1 -> Max/2
  Abs/1 -> Max/1
  Add2/1 -> Abs2/1
  Add1/1 -> Abs1/1
  Add/1 -> Abs/1
  Demux/3 -> Add2/1
  Demux1/3 -> Add2/2
  Demux1/2 -> Add1/2
  Demux/2 -> Add1/1
  Demux1/1 -> Add/2
  Demux/1 -> Add/1
  v000_k_1/1 -> Demux1/1
  v222_k_1/1 -> Demux/1

== system ASEToolBox/Subsystem/Formation-Control/Follower2/Subsystem1 ==
  Clock : Clock
  Constant : Constant
  Constant1 : Constant  Value=0
  Switch1 : Switch  Criteria=u2 > Threshold  Threshold=40  SaturateOnIntegerOverflow=off  InputSameDT=off
  Out1 : Outport
  wires:
  Clock/1 -> Switch1/2
  Constant/1 -> Switch1/1
  Constant1/1 -> Switch1/3
  Switch1/1 -> Out1/1

== system ASEToolBox/Subsystem/Formation-Control/Follower2/质心运动方程 ==
  v2 : Inport
  theta2 : Inport  Port=2
  phi2 : Inport  Port=3
  Enable : EnablePort
  Cos : Trigonometry  Operator=cos
  Cos1 : Trigonometry  Operator=cos
  Mux : Mux  Inputs=3
  Product : Product  Inputs=3
  Product1 : Product  Inputs=3
  Product2 : Product
  Sin : Trigonometry
  Sin1 : Trigonometry
  v222 : Outport
  wires:
  theta2/1 -> Cos/1, Sin/1
  phi2/1 -> Cos1/1, Sin1/1
  Cos/1 -> Product/1
  v2/1 -> Product2/2, Product1/3, Product/3
  Product/1 -> Mux/1
  Product1/1 -> Mux/2
  Sin/1 -> Product1/1
  Cos1/1 -> Product/2, Product1/2
  Product2/1 -> Mux/3
  Mux/1 -> v222/1
  Sin1/1 -> Product2/1

== system ASEToolBox/Subsystem/Formation-Control/Follower3/Subsystem ==
  v333_k_1 : Inport
  v000_k_1 : Inport  Port=2
  Abs : Abs  SaturateOnIntegerOverflow=off
  Abs1 : Abs  SaturateOnIntegerOverflow=off
  Abs2 : Abs  SaturateOnIntegerOverflow=off
  Add : Sum  Inputs=+-
  Add1 : Sum  Inputs=+-
  Add2 : Sum  Inputs=+-
  Demux : Demux  Outputs=3
  Demux1 : Demux  Outputs=3
  Max : MinMax  Function=max  Inputs=3
  Relational Operator : RelationalOperator  Operator=>  OutDataTypeStr=boolean  RndMeth=Simplest  InputSameDT=off
  get lmd : Subsystem
  order : Outport
  wires:
  v333_k_1/1 -> Demux/1
  v000_k_1/1 -> Demux1/1
  Demux/1 -> Add/1
  Demux1/1 -> Add/2
  Demux/2 -> Add1/1
  Demux1/2 -> Add1/2
  Demux1/3 -> Add2/2
  Demux/3 -> Add2/1
  Add/1 -> Abs/1
  Add1/1 -> Abs1/1
  Add2/1 -> Abs2/1
  Abs/1 -> Max/1
  Abs1/1 -> Max/2
  Abs2/1 -> Max/3
  Max/1 -> Relational Operator/1
  get lmd/1(lmd) -> Relational Operator/2
  Relational Operator/1 -> order/1

== system ASEToolBox/Subsystem/Formation-Control/Follower3/Subsystem1 ==
  Clock : Clock
  Constant : Constant
  Constant1 : Constant  Value=0
  Switch1 : Switch  Criteria=u2 > Threshold  Threshold=40  SaturateOnIntegerOverflow=off  InputSameDT=off
  Out1 : Outport
  wires:
  Clock/1 -> Switch1/2
  Constant/1 -> Switch1/1
  Constant1/1 -> Switch1/3
  Switch1/1 -> Out1/1

== system ASEToolBox/Subsystem/Formation-Control/Follower3/质心运动方程 ==
  v3 : Inport
  theta3 : Inport  Port=2
  phi3 : Inport  Port=3
  Enable : EnablePort
  Cos : Trigonometry  Operator=cos
  Cos1 : Trigonometry  Operator=cos
  Mux : Mux  Inputs=3
  Product : Product  Inputs=3
  Product1 : Product  Inputs=3
  Product2 : Product
  Sin : Trigonometry
  Sin1 : Trigonometry
  v333 : Outport
  wires:
  Sin1/1 -> Product2/1
  Mux/1 -> v333/1
  Product2/1 -> Mux/3
  Cos1/1 -> Product1/2, Product/2
  Sin/1 -> Product1/1
  Product1/1 -> Mux/2
  Product/1 -> Mux/1
  v3/1 -> Product/3, Product1/3, Product2/2
  Cos/1 -> Product/1
  phi3/1 -> Sin1/1, Cos1/1
  theta3/1 -> Sin/1, Cos/1

== system ASEToolBox/Subsystem/Formation-Control/Leader/W0-Φ ==
  Digital Clock : DigitalClock  SampleTime=dt
  Gain1 : Gain  Gain=0.2
  Gain2 : Gain  Gain=0.1
  Sin : Trigonometry  Operator=cos
  W0 : Outport
  wires:
  Digital Clock/1 -> Gain1/1
  Gain1/1 -> Sin/1
  Sin/1 -> Gain2/1
  Gain2/1 -> W0/1

== system ASEToolBox/Subsystem/Formation-Control/Leader/r0-v ==
  Digital Clock : DigitalClock  SampleTime=dt
  Gain1 : Gain  Gain=0.4
  Gain2 : Gain  Gain=0.1
  Scope : Scope
      settings: ActiveDisplayYMinimum=-0.125  ActiveDisplayYMaximum=0.125
  Sin : Trigonometry
  r0 : Outport
  wires:
  Digital Clock/1 -> Gain1/1
  Gain1/1 -> Sin/1
  Sin/1 -> Gain2/1
  Gain2/1 -> Scope/1, r0/1

== system ASEToolBox/Subsystem/Formation-Control/Leader/w0-θ ==
  Digital Clock : DigitalClock  SampleTime=dt
  Gain1 : Gain  Gain=0.2
  Gain2 : Gain  Gain=0.1
  Sin : Trigonometry  Operator=cos
  w0 : Outport
  wires:
  Gain2/1 -> w0/1
  Sin/1 -> Gain2/1
  Gain1/1 -> Sin/1
  Digital Clock/1 -> Gain1/1

== system ASEToolBox/Subsystem/Formation-Control/Leader/质心运动方程 ==
  theta0 : Inport
  phi0 : Inport  Port=2
  v0 : Inport  Port=3
  Cos : Trigonometry  Operator=cos
  Cos1 : Trigonometry  Operator=cos
  Mux : Mux  Inputs=3
  Product : Product  Inputs=3
  Product1 : Product  Inputs=3
  Product2 : Product
  Sin : Trigonometry
  Sin1 : Trigonometry
  v000 : Outport
  wires:
  theta0/1 -> Cos/1, Sin/1
  phi0/1 -> Sin1/1, Cos1/1
  Cos/1 -> Product/1
  v0/1 -> Product2/2, Product1/3, Product/3
  Product/1 -> Mux/1
  Product1/1 -> Mux/2
  Sin/1 -> Product1/1
  Cos1/1 -> Product1/2, Product/2
  Product2/1 -> Mux/3
  Mux/1 -> v000/1
  Sin1/1 -> Product2/1

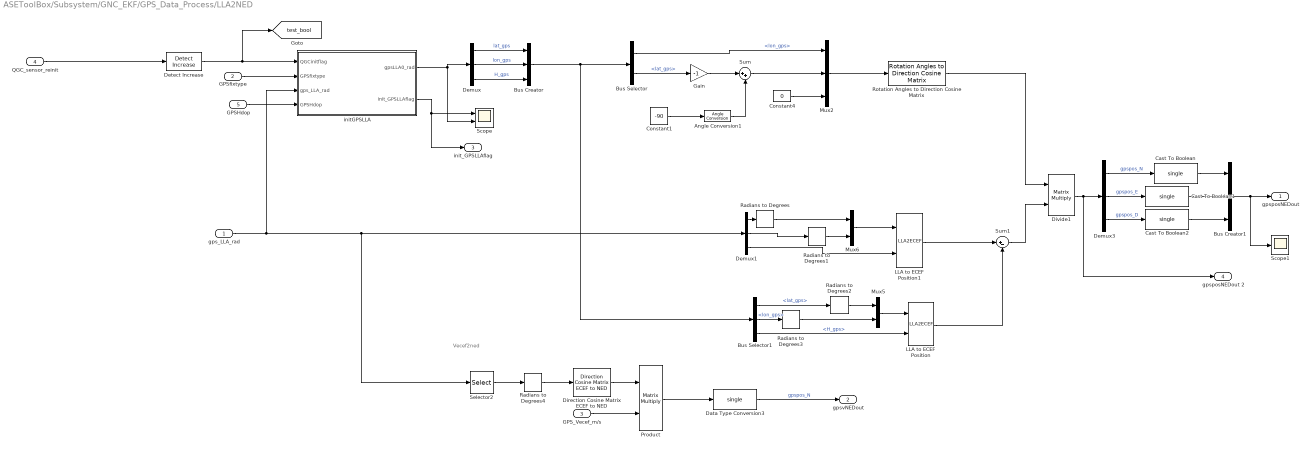
== system ASEToolBox/Subsystem/GNC_EKF/GPS_Data_Process/LLA2NED ==
  note: Vecef2ned
  gps_LLA_rad : Inport
  GPSfixtype : Inport  Port=2
  GPS_Vecef_m/s : Inport  Port=3
  QGC_sensor_reinit : Inport  Port=4
  GPSHdop : Inport  Port=5
  Angle Conversion1 : aerolibconvert2/Angle Conversion  IU=deg  OU=rad
  Bus Creator : BusCreator  Inputs=3
  Bus Creator1 : BusCreator  Inputs=3
  Bus Selector : BusSelector  OutputSignals=lon_gps,lat_gps
  Bus Selector1 : BusSelector  OutputSignals=lat_gps,lon_gps,H_gps
  Cast To Boolean : DataTypeConversion  OutDataTypeStr=single  SaturateOnIntegerOverflow=off  RndMeth=Floor
  Cast To Boolean1 : DataTypeConversion  OutDataTypeStr=single  SaturateOnIntegerOverflow=off  RndMeth=Floor
  Cast To Boolean2 : DataTypeConversion  OutDataTypeStr=single  SaturateOnIntegerOverflow=off  RndMeth=Floor
  Constant1 : Constant  Value=-90
  Constant4 : Constant  Value=0
  Data Type Conversion3 : DataTypeConversion  OutDataTypeStr=single  SaturateOnIntegerOverflow=off  RndMeth=Floor
  Demux : Demux  Outputs=3
  Demux1 : Demux  Outputs=3
  Demux3 : Demux  Outputs=3
  Detect Increase : simulink/Logic and Bit Operations/Detect Increase  vinit=0.0  OutDataTypeStr=boolean
  Direction Cosine Matrix ECEF to NED : aerolibtransform2/Direction Cosine Matrix ECEF to NED
  Divide1 : Product  Inputs=**  Multiplication=Matrix(*)
  Gain : Gain  Gain=-1
  LLA to ECEF Position : LLA2ECEF  R=6378137
  LLA to ECEF Position1 : LLA2ECEF  R=6378137
  Mux2 : Mux  Inputs=3
  Mux5 : Mux  Inputs=2
  Mux6 : Mux  Inputs=2
  Product : Product  Multiplication=Matrix(*)
  Radians to Degrees{,1..4} (5 alike) : simulink_extras/Transformations/Radians to Degrees
  Rotation Angles to Direction Cosine Matrix : sharedtransform/Rotation Angles to Direction Cosine Matrix  rotationOrder=ZYX  aMode=aMode
  Scope : Scope  NumInputPorts=2
      settings: ActiveDisplayYMinimum=-1  ActiveDisplayYMaximum=1  DataLoggingVariableName=ScopeData2
  Scope1 : Scope
      settings: ActiveDisplayYMinimum=-15.73235  ActiveDisplayYMaximum=8.44126  DataLoggingVariableName=ScopeData8
  Selector2 : Selector  InputPortWidth=3  IndexOptions=Index vector (dialog)  Indices=[1 2]  OutputSizes=1
  Sum : Sum  Inputs=|++
  Sum1 : Sum  Inputs=|+-
  initGPSLLA : MATLAB Function  TreatAsAtomicUnit=on
  "gpsposNEDout " : Outport
  gpsvNEDout : Outport  Port=2
  init_GPSLLAflag : Outport  Port=3
  gpsposNEDout 2 : Outport  Port=4
  tag scope: test_bool=global
  wires:
  GPSfixtype/1 -> initGPSLLA/2(GPSfixtype)
  Bus Creator1/1 -> Scope1/1, "gpsposNEDout "/1
  Demux3/3 -> Cast To Boolean2/1  "gpspos_D"
  Demux3/2 -> Cast To Boolean1/1  "gpspos_E"
  Demux3/1 -> Cast To Boolean/1  "gpspos_N"
  Bus Creator/1 -> Bus Selector/1, Bus Selector1/1
  Demux/3 -> Bus Creator/3  "H_gps"
  Demux/2 -> Bus Creator/2  "lon_gps"
  Demux/1 -> Bus Creator/1  "lat_gps"
  Demux1/3 -> LLA to ECEF Position1/2
  Mux6/1 -> LLA to ECEF Position1/1
  Mux5/1 -> LLA to ECEF Position/1
  Gain/1 -> Sum/1
  LLA to ECEF Position1/1 -> Sum1/1
  Constant4/1 -> Mux2/3
  Sum1/1 -> Divide1/2
  Divide1/1 -> gpsposNEDout 2/1, Demux3/1
  Demux1/1 -> Radians to Degrees/1
  Mux2/1 -> Rotation Angles to Direction Cosine Matrix/1
  Rotation Angles to Direction Cosine Matrix/1 -> Divide1/1
  Constant1/1 -> Angle Conversion1/1
  LLA to ECEF Position/1 -> Sum1/2
  Demux1/2 -> Radians to Degrees1/1
  Sum/1 -> Mux2/2
  Bus Selector/2 -> Gain/1  "<lat_gps>"
  Bus Selector/1 -> Mux2/1  "<lon_gps>"
  Bus Selector1/1 -> Radians to Degrees2/1  "<lat_gps>"
  Bus Selector1/2 -> Radians to Degrees3/1  "<lon_gps>"
  Bus Selector1/3 -> LLA to ECEF Position/2  "<H_gps>"
  gps_LLA_rad/1 -> initGPSLLA/3(gps_LLA_rad), Selector2/1, Demux1/1
  Radians to Degrees/1 -> Mux6/1
  Radians to Degrees1/1 -> Mux6/2
  Angle Conversion1/1 -> Sum/2
  Radians to Degrees2/1 -> Mux5/1
  Radians to Degrees3/1 -> Mux5/2
  GPS_Vecef_m/s/1 -> Product/2
  Direction Cosine Matrix ECEF to NED/1 -> Product/1
  Selector2/1 -> Radians to Degrees4/1
  Radians to Degrees4/1 -> Direction Cosine Matrix ECEF to NED/1
  Data Type Conversion3/1 -> gpsvNEDout/1  "gpspos_N"
  Detect Increase/1 -> [test_bool], initGPSLLA/1(QGCinitflag)
  initGPSLLA/1(gpsLLA0_rad) -> Demux/1, Scope/2
  initGPSLLA/2(init_GPSLLAflag) -> init_GPSLLAflag/1, Scope/1
  GPSHdop/1 -> initGPSLLA/4(GPSHdop)
  Cast To Boolean/1 -> Bus Creator1/1
  Cast To Boolean1/1 -> Bus Creator1/2
  Cast To Boolean2/1 -> Bus Creator1/3
  QGC_sensor_reinit/1 -> Detect Increase/1
  Product/1 -> Data Type Conversion3/1

== system ASEToolBox/Subsystem/GNC_EKF/GPS_Data_Process/TD_baro ==
  H_baro : Inport
  Constant1 : Constant  Value=0.002  OutDataTypeStr=double
  Constant3 : Constant  Value=0.23  OutDataTypeStr=double
  Constant4 : Constant  Value=900  OutDataTypeStr=single
  Data Type Conversion : DataTypeConversion  OutDataTypeStr=single  SaturateOnIntegerOverflow=off  RndMeth=Floor
  Data Type Conversion1 : DataTypeConversion  OutDataTypeStr=single  SaturateOnIntegerOverflow=off  RndMeth=Floor
  Data Type Conversion5 : DataTypeConversion  OutDataTypeStr=single  SaturateOnIntegerOverflow=off  RndMeth=Floor
  Delay1 : Delay  DelayLength=1  InitialConditionSource=Input port
      settings: InputPortMap=u0,p4
  MATLAB Function2 : MATLAB Function  TreatAsAtomicUnit=on
  Memory : Memory  InheritSampleTime=on
  Scope : Scope  NumInputPorts=3
      settings: ActiveDisplayYMinimum=-89.45584  ActiveDisplayYMaximum=789.64981
  vH_baro_TD : Outport
  H_baro_TD : Outport  Port=2
  wires:
  Delay1/1 -> H_baro_TD/1, Scope/3, MATLAB Function2/3("u1 ")
  H_baro/1 -> Data Type Conversion5/1
  Memory/1 -> MATLAB Function2/4("u2 "), vH_baro_TD/1, Scope/2
  Constant3/1 -> Data Type Conversion1/1
  Constant4/1 -> MATLAB Function2/6(r)
  MATLAB Function2/1(u1) -> Delay1/1
  MATLAB Function2/2(u2) -> Memory/1
  Data Type Conversion5/1 -> Scope/1, Delay1/2, MATLAB Function2/2(u0)
  Constant1/1 -> Data Type Conversion/1
  Data Type Conversion/1 -> MATLAB Function2/1(T)
  Data Type Conversion1/1 -> MATLAB Function2/5(h)

== system ASEToolBox/Subsystem/GNC_EKF/GPS_Data_Process/TD_baro1 ==
  H_baro : Inport
  Constant1 : Constant  Value=0.002  OutDataTypeStr=double
  Constant3 : Constant  Value=0.23  OutDataTypeStr=double
  Constant4 : Constant  Value=900  OutDataTypeStr=single
  Data Type Conversion : DataTypeConversion  OutDataTypeStr=single  SaturateOnIntegerOverflow=off  RndMeth=Floor
  Data Type Conversion1 : DataTypeConversion  OutDataTypeStr=single  SaturateOnIntegerOverflow=off  RndMeth=Floor
  Data Type Conversion5 : DataTypeConversion  OutDataTypeStr=single  SaturateOnIntegerOverflow=off  RndMeth=Floor
  Delay1 : Delay  DelayLength=1  InitialConditionSource=Input port
      settings: InputPortMap=u0,p4
  MATLAB Function2 : MATLAB Function  TreatAsAtomicUnit=on
  Memory : Memory  InheritSampleTime=on
  Scope : Scope  NumInputPorts=3
      settings: ActiveDisplayYMinimum=-89.45584  ActiveDisplayYMaximum=789.64981
  vH_baro_TD : Outport
  H_baro_TD : Outport  Port=2
  wires:
  Data Type Conversion5/1 -> MATLAB Function2/2(u0), Delay1/2, Scope/1
  MATLAB Function2/2(u2) -> Memory/1
  MATLAB Function2/1(u1) -> Delay1/1
  Constant4/1 -> MATLAB Function2/6(r)
  Constant1/1 -> Data Type Conversion/1
  Constant3/1 -> Data Type Conversion1/1
  Memory/1 -> Scope/2, vH_baro_TD/1, MATLAB Function2/4("u2 ")
  H_baro/1 -> Data Type Conversion5/1
  Delay1/1 -> MATLAB Function2/3("u1 "), Scope/3, H_baro_TD/1
  Data Type Conversion/1 -> MATLAB Function2/1(T)
  Data Type Conversion1/1 -> MATLAB Function2/5(h)
